simulink model "pivotsimulation"  (R2026a)
settings: Solver=ode15s  StopTime=30  AbsTol=1e-3  EnableMultiTasking=on
undefined symbols (not defined in the file): X, Y, Z
libraries: sm_lib x21, nesl_utility x4
settings Model: Creator=emmak  LastModifiedBy=emmak
settings DebuggingCC: SubsystemReferenceDiagnosticForUnitTest=warning
settings SimscapeCC: SimscapeNominalValues="[{\"value\":\"1\",\"unit\":\"A\"},{\"value\":\"1\",\"unit\":\"bar\"},{\"value\":\"1\",\"unit\":\"cm^2\"},{\"value\":\"1\",\"unit\":\"cm^3/s\"},{\"value\":\"1\",\"unit\":\"kJ/kg\"},{\"value\":\"1\",\"unit\":\"kW\"},{\"value\":\"1\",\"unit\":\"l\"},{\"value\":\"1\",\"unit\":\"N\"},{\"value\":\"1\",\"unit\":\"N*m\"},{\"value\":\"1\",\"unit\":\"V\"}]"

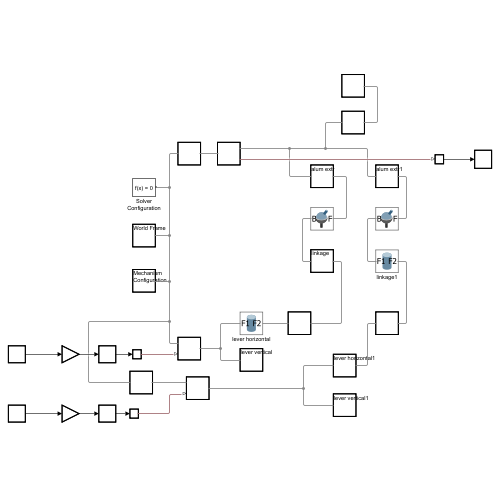
[thumbnail: Simulink's stored preview of the top-level diagram]
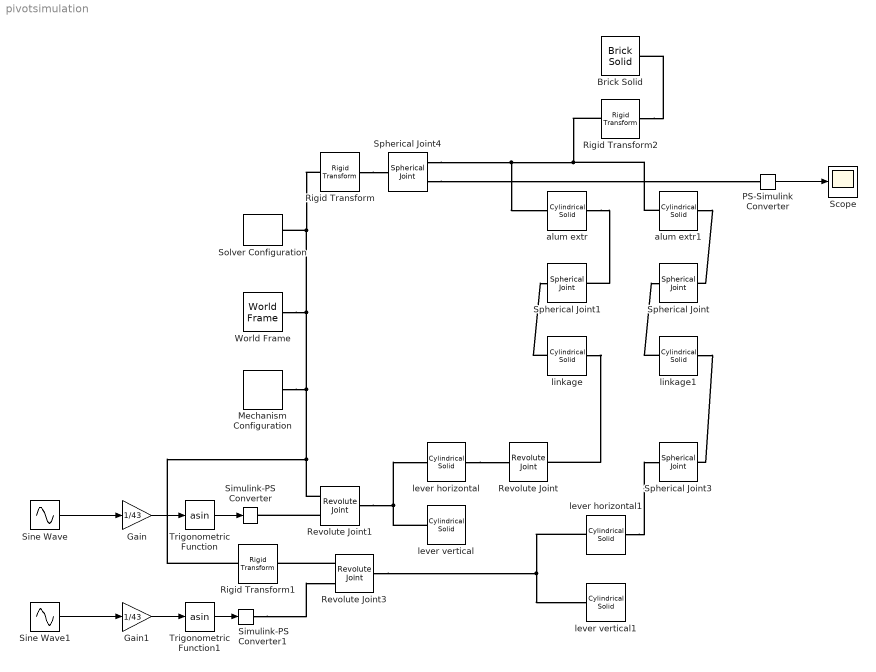
== system pivotsimulation ==
  Brick Solid : sm_lib/Body Elements/Brick Solid  BrickDimensions=[600 10 400]  BrickDimensionsUnits=mm  ExportEntireGeometry=off  InertiaType=CalculateFromGeometry  BasedOnType=Density  Density=1000  DensityUnits=kg/m^3  Mass=1  MassUnits=kg  CenterOfMass=[0 0 0]  CenterOfMassUnits=m  MomentsOfInertia=[1 1 1]  MomentsOfInertiaUnits=kg*m^2  ProductsOfInertia=[0 0 0]  ProductsOfInertiaUnits=kg*m^2  GraphicType=FromGeometry  MarkerShape=Sphere  MarkerSize=10  GraphicVisPropType=SimpleVisualProperties  GraphicDiffuseColor=[0.6471 0.5255 0.3843]  GraphicOpacity=1  GraphicSpecularColor=[0.5 0.5 0.5 1.0]  GraphicAmbientColor=[0.15 0.15 0.15 1.0]  GraphicEmissiveColor=[0.0 0.0 0.0 1.0]  GraphicShininess=75  DoExposeReferenceFrame=on  SerializedFrames=<Frames/>
  Gain : Gain  Gain=1/43
  Gain1 : Gain  Gain=1/43
  Mechanism Configuration : sm_lib/Utilities/Mechanism Configuration  UniformGravity=Constant  GravityVector=[0 -9.80665 0]  GravityVectorUnits=m/s^2  LinearizationDelta=0.001  JointModeTransitionNonlinearIterations=2
  PS-Simulink Converter : nesl_utility/PS-Simulink Converter  PhysicalDomain=network_engine_domain  SubClassName=ps_output  LeftPortType=input  RightPortType=output  PseudoPeriodic=off  Frequencies=[]  VectorFormat=inherit  Unit=inherit  AffineConversion=off
  Revolute Joint : sm_lib/Joints/Revolute Joint  JointMode=Normal  CompositeWrenchDir=FollowerOnBase  CompositeWrenchFrame=BaseFrame  SenseConstraintForce=off  SenseConstraintTorque=off  SenseTotalForce=off  SenseTotalTorque=off  PositionTargetSpecify=off  PositionTargetPriority=High  PositionTargetValue=0  PositionTargetValueUnits=deg  VelocityTargetSpecify=off  VelocityTargetPriority=High  VelocityTargetValue=0  VelocityTargetValueUnits=deg/s  EquilibriumPosition=0  EquilibriumPositionUnits=deg  SpringStiffness=0  SpringStiffnessUnits=N*m/deg  DampingCoefficient=0  DampingCoefficientUnits=N*m/(deg/s)  LowerLimitSpecify=off  LowerLimitBound=-90  LowerLimitBoundUnits=deg  LowerLimitStiffness=1e4  LowerLimitStiffnessUnits=N*m/deg  LowerLimitDamping=10  LowerLimitDampingUnits=N*m/(deg/s)  LowerLimitTransitionRegionWidth=0.1  LowerLimitTransitionRegionWidthUnits=deg  UpperLimitSpecify=off  UpperLimitBound=90  UpperLimitBoundUnits=deg  UpperLimitStiffness=1e4  UpperLimitStiffnessUnits=N*m/deg  UpperLimitDamping=10  UpperLimitDampingUnits=N*m/(deg/s)  UpperLimitTransitionRegionWidth=0.1  UpperLimitTransitionRegionWidthUnits=deg  TorqueActuationMode=NoTorque  MotionActuationMode=ComputedMotion  SensePosition=off  SenseVelocity=off  SenseAcceleration=off  SenseTorqueForce=off  SenseLowerLimitTorqueForce=off  SenseUpperLimitTorqueForce=off
  Revolute Joint1 : sm_lib/Joints/Revolute Joint  JointMode=Normal  CompositeWrenchDir=FollowerOnBase  CompositeWrenchFrame=BaseFrame  SenseConstraintForce=off  SenseConstraintTorque=off  SenseTotalForce=off  SenseTotalTorque=off  PositionTargetSpecify=off  PositionTargetPriority=High  PositionTargetValue=0  PositionTargetValueUnits=deg  VelocityTargetSpecify=off  VelocityTargetPriority=High  VelocityTargetValue=0  VelocityTargetValueUnits=deg/s  EquilibriumPosition=0  EquilibriumPositionUnits=deg  SpringStiffness=0  SpringStiffnessUnits=N*m/deg  DampingCoefficient=0  DampingCoefficientUnits=N*m/(deg/s)  LowerLimitSpecify=off  LowerLimitBound=-90  LowerLimitBoundUnits=deg  LowerLimitStiffness=1e4  LowerLimitStiffnessUnits=N*m/deg  LowerLimitDamping=10  LowerLimitDampingUnits=N*m/(deg/s)  LowerLimitTransitionRegionWidth=0.1  LowerLimitTransitionRegionWidthUnits=deg  UpperLimitSpecify=off  UpperLimitBound=90  UpperLimitBoundUnits=deg  UpperLimitStiffness=1e4  UpperLimitStiffnessUnits=N*m/deg  UpperLimitDamping=10  UpperLimitDampingUnits=N*m/(deg/s)  UpperLimitTransitionRegionWidth=0.1  UpperLimitTransitionRegionWidthUnits=deg  TorqueActuationMode=ComputedTorque  MotionActuationMode=InputMotion  SensePosition=off  SenseVelocity=off  SenseAcceleration=off  SenseTorqueForce=off  SenseLowerLimitTorqueForce=off  SenseUpperLimitTorqueForce=off
  Revolute Joint3 : sm_lib/Joints/Revolute Joint  JointMode=Normal  CompositeWrenchDir=FollowerOnBase  CompositeWrenchFrame=BaseFrame  SenseConstraintForce=off  SenseConstraintTorque=off  SenseTotalForce=off  SenseTotalTorque=off  PositionTargetSpecify=off  PositionTargetPriority=High  PositionTargetValue=0  PositionTargetValueUnits=deg  VelocityTargetSpecify=off  VelocityTargetPriority=High  VelocityTargetValue=0  VelocityTargetValueUnits=deg/s  EquilibriumPosition=0  EquilibriumPositionUnits=deg  SpringStiffness=0  SpringStiffnessUnits=N*m/deg  DampingCoefficient=0  DampingCoefficientUnits=N*m/(deg/s)  LowerLimitSpecify=off  LowerLimitBound=-90  LowerLimitBoundUnits=deg  LowerLimitStiffness=1e4  LowerLimitStiffnessUnits=N*m/deg  LowerLimitDamping=10  LowerLimitDampingUnits=N*m/(deg/s)  LowerLimitTransitionRegionWidth=0.1  LowerLimitTransitionRegionWidthUnits=deg  UpperLimitSpecify=off  UpperLimitBound=90  UpperLimitBoundUnits=deg  UpperLimitStiffness=1e4  UpperLimitStiffnessUnits=N*m/deg  UpperLimitDamping=10  UpperLimitDampingUnits=N*m/(deg/s)  UpperLimitTransitionRegionWidth=0.1  UpperLimitTransitionRegionWidthUnits=deg  TorqueActuationMode=ComputedTorque  MotionActuationMode=InputMotion  SensePosition=off  SenseVelocity=off  SenseAcceleration=off  SenseTorqueForce=off  SenseLowerLimitTorqueForce=off  SenseUpperLimitTorqueForce=off
  Rigid Transform : sm_lib/Frames and Transforms/Rigid Transform  RotationMethod=None  FollAlignAxisA=+X  BaseAlignAxisA=+Y  FollAlignAxisB=+Y  BaseAlignAxisB=+Z  RotationStandardAxis=+Z  RotationAngle=0  RotationAngleUnits=deg  RotationArbitraryAxis=[0 0 1]  RotationSequenceAxes=FollowerAxes  RotationSequence=XYX  RotationSequenceAngles=[0 0 0]  RotationSequenceAnglesUnits=deg  RotationMatrix=[1 0 0;0 1 0;0 0 1]  Quaternion=[1 0 0 0]  TranslationMethod=Cartesian  TranslationCartesianOffset=[265 91 0]  TranslationCartesianOffsetUnits=mm  TranslationStandardAxis=+Z  TranslationStandardOffset=0  TranslationStandardOffsetUnits=m  TranslationROffset=0  TranslationROffsetUnits=m  TranslationThetaOffset=0  TranslationThetaOffsetUnits=deg  TranslationZOffset=0  TranslationZOffsetUnits=m
  Rigid Transform1 : sm_lib/Frames and Transforms/Rigid Transform  RotationMethod=None  FollAlignAxisA=+X  BaseAlignAxisA=+Y  FollAlignAxisB=+Y  BaseAlignAxisB=+Z  RotationStandardAxis=+Z  RotationAngle=0  RotationAngleUnits=deg  RotationArbitraryAxis=[0 0 1]  RotationSequenceAxes=FollowerAxes  RotationSequence=XYX  RotationSequenceAngles=[0 0 0]  RotationSequenceAnglesUnits=deg  RotationMatrix=[1 0 0;0 1 0;0 0 1]  Quaternion=[1 0 0 0]  TranslationMethod=Cartesian  TranslationCartesianOffset=[285 0 146]  TranslationCartesianOffsetUnits=mm  TranslationStandardAxis=+Z  TranslationStandardOffset=0  TranslationStandardOffsetUnits=m  TranslationROffset=0  TranslationROffsetUnits=m  TranslationThetaOffset=0  TranslationThetaOffsetUnits=deg  TranslationZOffset=0  TranslationZOffsetUnits=m
  Rigid Transform2 : sm_lib/Frames and Transforms/Rigid Transform  RotationMethod=None  FollAlignAxisA=+X  BaseAlignAxisA=+Y  FollAlignAxisB=+Y  BaseAlignAxisB=+Z  RotationStandardAxis=+Z  RotationAngle=0  RotationAngleUnits=deg  RotationArbitraryAxis=[0 0 1]  RotationSequenceAxes=FollowerAxes  RotationSequence=XYX  RotationSequenceAngles=[0 0 0]  RotationSequenceAnglesUnits=deg  RotationMatrix=[1 0 0;0 1 0;0 0 1]  Quaternion=[1 0 0 0]  TranslationMethod=Cartesian  TranslationCartesianOffset=[0 10 0]  TranslationCartesianOffsetUnits=mm  TranslationStandardAxis=+Z  TranslationStandardOffset=0  TranslationStandardOffsetUnits=m  TranslationROffset=0  TranslationROffsetUnits=m  TranslationThetaOffset=0  TranslationThetaOffsetUnits=deg  TranslationZOffset=0  TranslationZOffsetUnits=m
  Scope : Scope
      settings: ActiveDisplayYMinimum=-0.3302984984477686  ActiveDisplayYMaximum=0.32500944706024004
  Simulink-PS Converter : nesl_utility/Simulink-PS Converter  PhysicalDomain=network_engine_domain  SubClassName=ps_input  LeftPortType=input  RightPortType=output  PseudoPeriodic=off  Frequencies=[]  NoiseDistribution=none  NoiseParameters=[]  Unit=1  AffineConversion=off  FilteringAndDerivatives=filter  SimscapeFilterOrder=2  InputFilterTimeConstant=0.001  UdotUserProvided=0
  Simulink-PS Converter1 : nesl_utility/Simulink-PS Converter  PhysicalDomain=network_engine_domain  SubClassName=ps_input  LeftPortType=input  RightPortType=output  PseudoPeriodic=off  Frequencies=[]  NoiseDistribution=none  NoiseParameters=[]  Unit=1  AffineConversion=off  FilteringAndDerivatives=filter  SimscapeFilterOrder=2  InputFilterTimeConstant=0.001  UdotUserProvided=0
  Sine Wave : Sin  Amplitude=25  SampleTime=0
  Sine Wave1 : Sin  Amplitude=25  Frequency=1.5  Phase=(pi)  SampleTime=0
  Solver Configuration : nesl_utility/Solver Configuration  PhysicalDomain=network_engine_domain  SubClassName=solver  LeftPortType=input  RightPortType=generic  Tones=[]  Harmonics=[]  SimulateNoise=off  Profile=off  UseLocalSampling=off  EnableSwitchedLinearOptims=on  FrequencyDomain=off  UseCCode=off  RelTol=0.001  AbsTol=1e-06  MinStep=1e-09  ToWorkspace=off  RevertToSquareIcSolve=off  NumHomotopyIterations=100  PhasorMode=off  PhasorModeNumHarmonics=1  ConsistencySolver=NEWTON_XTOL_AFTER_FTOL  CanonicalOrdering=UNORDERED  OptimizeIntermediates=UNOPTIMIZED  IndexReductionMethod=DerivativeReplacement  DoDC=off  ResidualTolerance=1e-09  ConsistencyTolSource=GLOBAL  ConsistencyAbsTol=0.001  ConsistencyRelTol=0.001  ConsistencyTolFactor=0.001  UseLocalSolver=off  LocalSolverChoice=NE_BACKWARD_EULER_ADVANCER  ResolveIndetEquations=on  FunctionEvalNumThread=1  LocalSolverSampleTime=0.001  DoFixedCost=off  MaxNonlinIter=3  MaxModeIter=2  ComputeImpulses=off  ImpulseIterations=2  LinearAlgebra=Sparse  LinearAlgebraNumThread=0  EquationFormulation=NE_TIME_EF  DelaysMemoryBudget=1024  AutomaticFiltering=on  FilteringTimeConstant=0.001  PartitionStorageMethod=AS_NEEDED  PartitionMemoryBudget=1024  PartitionMethod=FAST  MultibodyUseLocalSolver=off  MultibodyLocalSolverChoice=ODE1  MultibodyLocalSolverSampleTime=0.001
  Spherical Joint : sm_lib/Joints/Spherical Joint  JointMode=Normal  CompositeWrenchDir=FollowerOnBase  CompositeWrenchFrame=BaseFrame  SenseConstraintForce=off  SenseConstraintTorque=off  SenseTotalForce=off  SenseTotalTorque=off  PositionTargetSpecify=off  PositionTargetPriority=High  PositionTargetRotationMethod=None  PositionTargetFollAlignAxisA=+X  PositionTargetBaseAlignAxisA=+Y  PositionTargetFollAlignAxisB=+Y  PositionTargetBaseAlignAxisB=+Z  PositionTargetRotationStandardAxis=+Z  PositionTargetRotationAngle=0  PositionTargetRotationAngleUnits=deg  PositionTargetRotationArbitraryAxis=[0 0 1]  PositionTargetRotationSequenceAxes=FollowerAxes  PositionTargetRotationSequence=XYX  PositionTargetRotationSequenceAngles=[0 0 0]  PositionTargetRotationSequenceAnglesUnits=deg  PositionTargetRotationMatrix=[1 0 0;0 1 0;0 0 1]  PositionTargetQuaternion=[1 0 0 0]  VelocityTargetSpecify=off  VelocityTargetPriority=High  VelocityTargetValue=[0 0 0]  VelocityTargetValueUnits=deg/s  VelocityTargetInFollowerFrame=on  EqPosRotationMethod=None  EqPosFollAlignAxisA=+X  EqPosBaseAlignAxisA=+Y  EqPosFollAlignAxisB=+Y  EqPosBaseAlignAxisB=+Z  EqPosRotationStandardAxis=+Z  EqPosRotationAngle=0  EqPosRotationAngleUnits=deg  EqPosRotationArbitraryAxis=[0 0 1]  EqPosRotationSequenceAxes=FollowerAxes  EqPosRotationSequence=XYX  EqPosRotationSequenceAngles=[0 0 0]  EqPosRotationSequenceAnglesUnits=deg  EqPosRotationMatrix=[1 0 0;0 1 0;0 0 1]  EqPosQuaternion=[1 0 0 0]  SpringStiffness=0  SpringStiffnessUnits=N*m/deg  DampingCoefficient=0  DampingCoefficientUnits=N*m/(deg/s)  LowerLimitSpecify=off  LowerLimitBound=15  LowerLimitBoundUnits=deg  LowerLimitStiffness=1e4  LowerLimitStiffnessUnits=N*m/deg  LowerLimitDamping=10  LowerLimitDampingUnits=N*m/(deg/s)  LowerLimitTransitionRegionWidth=0.1  LowerLimitTransitionRegionWidthUnits=deg  UpperLimitSpecify=off  UpperLimitBound=45  UpperLimitBoundUnits=deg  UpperLimitStiffness=1e4  UpperLimitStiffnessUnits=N*m/deg  UpperLimitDamping=10  UpperLimitDampingUnits=N*m/(deg/s)  UpperLimitTransitionRegionWidth=0.1  UpperLimitTransitionRegionWidthUnits=deg  TorqueActuationMode=NoTorque  ActuateTorqueX=off  ActuateTorqueY=off  ActuateTorqueZ=off  ActuateTorque=off  ActuationFrame=BaseFrame  SensePosition=off  SenseVelocityX=off  SenseVelocityY=off  SenseVelocityZ=off  SenseVelocity=off  SenseAccelerationX=off  SenseAccelerationY=off  SenseAccelerationZ=off  SenseAcceleration=off  SenseLowerLimitTorqueMag=off  SenseUpperLimitTorqueMag=off  SensingFrame=BaseFrame
  Spherical Joint1 : sm_lib/Joints/Spherical Joint  JointMode=Normal  CompositeWrenchDir=FollowerOnBase  CompositeWrenchFrame=BaseFrame  SenseConstraintForce=off  SenseConstraintTorque=off  SenseTotalForce=off  SenseTotalTorque=off  PositionTargetSpecify=off  PositionTargetPriority=High  PositionTargetRotationMethod=None  PositionTargetFollAlignAxisA=+X  PositionTargetBaseAlignAxisA=+Y  PositionTargetFollAlignAxisB=+Y  PositionTargetBaseAlignAxisB=+Z  PositionTargetRotationStandardAxis=+Z  PositionTargetRotationAngle=0  PositionTargetRotationAngleUnits=deg  PositionTargetRotationArbitraryAxis=[0 0 1]  PositionTargetRotationSequenceAxes=FollowerAxes  PositionTargetRotationSequence=XYX  PositionTargetRotationSequenceAngles=[0 0 0]  PositionTargetRotationSequenceAnglesUnits=deg  PositionTargetRotationMatrix=[1 0 0;0 1 0;0 0 1]  PositionTargetQuaternion=[1 0 0 0]  VelocityTargetSpecify=off  VelocityTargetPriority=High  VelocityTargetValue=[0 0 0]  VelocityTargetValueUnits=deg/s  VelocityTargetInFollowerFrame=on  EqPosRotationMethod=None  EqPosFollAlignAxisA=+X  EqPosBaseAlignAxisA=+Y  EqPosFollAlignAxisB=+Y  EqPosBaseAlignAxisB=+Z  EqPosRotationStandardAxis=+Z  EqPosRotationAngle=0  EqPosRotationAngleUnits=deg  EqPosRotationArbitraryAxis=[0 0 1]  EqPosRotationSequenceAxes=FollowerAxes  EqPosRotationSequence=XYX  EqPosRotationSequenceAngles=[0 0 0]  EqPosRotationSequenceAnglesUnits=deg  EqPosRotationMatrix=[1 0 0;0 1 0;0 0 1]  EqPosQuaternion=[1 0 0 0]  SpringStiffness=0  SpringStiffnessUnits=N*m/deg  DampingCoefficient=0  DampingCoefficientUnits=N*m/(deg/s)  LowerLimitSpecify=off  LowerLimitBound=15  LowerLimitBoundUnits=deg  LowerLimitStiffness=1e4  LowerLimitStiffnessUnits=N*m/deg  LowerLimitDamping=10  LowerLimitDampingUnits=N*m/(deg/s)  LowerLimitTransitionRegionWidth=0.1  LowerLimitTransitionRegionWidthUnits=deg  UpperLimitSpecify=off  UpperLimitBound=45  UpperLimitBoundUnits=deg  UpperLimitStiffness=1e4  UpperLimitStiffnessUnits=N*m/deg  UpperLimitDamping=10  UpperLimitDampingUnits=N*m/(deg/s)  UpperLimitTransitionRegionWidth=0.1  UpperLimitTransitionRegionWidthUnits=deg  TorqueActuationMode=NoTorque  ActuateTorqueX=off  ActuateTorqueY=off  ActuateTorqueZ=off  ActuateTorque=off  ActuationFrame=BaseFrame  SensePosition=off  SenseVelocityX=off  SenseVelocityY=off  SenseVelocityZ=off  SenseVelocity=off  SenseAccelerationX=off  SenseAccelerationY=off  SenseAccelerationZ=off  SenseAcceleration=off  SenseLowerLimitTorqueMag=off  SenseUpperLimitTorqueMag=off  SensingFrame=BaseFrame
  Spherical Joint3 : sm_lib/Joints/Spherical Joint  JointMode=Normal  CompositeWrenchDir=FollowerOnBase  CompositeWrenchFrame=BaseFrame  SenseConstraintForce=off  SenseConstraintTorque=off  SenseTotalForce=off  SenseTotalTorque=off  PositionTargetSpecify=off  PositionTargetPriority=High  PositionTargetRotationMethod=None  PositionTargetFollAlignAxisA=+X  PositionTargetBaseAlignAxisA=+Y  PositionTargetFollAlignAxisB=+Y  PositionTargetBaseAlignAxisB=+Z  PositionTargetRotationStandardAxis=+Z  PositionTargetRotationAngle=0  PositionTargetRotationAngleUnits=deg  PositionTargetRotationArbitraryAxis=[0 0 1]  PositionTargetRotationSequenceAxes=FollowerAxes  PositionTargetRotationSequence=XYX  PositionTargetRotationSequenceAngles=[0 0 0]  PositionTargetRotationSequenceAnglesUnits=deg  PositionTargetRotationMatrix=[1 0 0;0 1 0;0 0 1]  PositionTargetQuaternion=[1 0 0 0]  VelocityTargetSpecify=off  VelocityTargetPriority=High  VelocityTargetValue=[0 0 0]  VelocityTargetValueUnits=deg/s  VelocityTargetInFollowerFrame=on  EqPosRotationMethod=None  EqPosFollAlignAxisA=+X  EqPosBaseAlignAxisA=+Y  EqPosFollAlignAxisB=+Y  EqPosBaseAlignAxisB=+Z  EqPosRotationStandardAxis=+Z  EqPosRotationAngle=0  EqPosRotationAngleUnits=deg  EqPosRotationArbitraryAxis=[0 0 1]  EqPosRotationSequenceAxes=FollowerAxes  EqPosRotationSequence=XYX  EqPosRotationSequenceAngles=[0 0 0]  EqPosRotationSequenceAnglesUnits=deg  EqPosRotationMatrix=[1 0 0;0 1 0;0 0 1]  EqPosQuaternion=[1 0 0 0]  SpringStiffness=0  SpringStiffnessUnits=N*m/deg  DampingCoefficient=0  DampingCoefficientUnits=N*m/(deg/s)  LowerLimitSpecify=off  LowerLimitBound=15  LowerLimitBoundUnits=deg  LowerLimitStiffness=1e4  LowerLimitStiffnessUnits=N*m/deg  LowerLimitDamping=10  LowerLimitDampingUnits=N*m/(deg/s)  LowerLimitTransitionRegionWidth=0.1  LowerLimitTransitionRegionWidthUnits=deg  UpperLimitSpecify=off  UpperLimitBound=45  UpperLimitBoundUnits=deg  UpperLimitStiffness=1e4  UpperLimitStiffnessUnits=N*m/deg  UpperLimitDamping=10  UpperLimitDampingUnits=N*m/(deg/s)  UpperLimitTransitionRegionWidth=0.1  UpperLimitTransitionRegionWidthUnits=deg  TorqueActuationMode=NoTorque  ActuateTorqueX=off  ActuateTorqueY=off  ActuateTorqueZ=off  ActuateTorque=off  ActuationFrame=BaseFrame  SensePosition=off  SenseVelocityX=off  SenseVelocityY=off  SenseVelocityZ=off  SenseVelocity=off  SenseAccelerationX=off  SenseAccelerationY=off  SenseAccelerationZ=off  SenseAcceleration=off  SenseLowerLimitTorqueMag=off  SenseUpperLimitTorqueMag=off  SensingFrame=BaseFrame
  Spherical Joint4 : sm_lib/Joints/Spherical Joint  JointMode=Normal  CompositeWrenchDir=FollowerOnBase  CompositeWrenchFrame=BaseFrame  SenseConstraintForce=off  SenseConstraintTorque=off  SenseTotalForce=off  SenseTotalTorque=off  PositionTargetSpecify=off  PositionTargetPriority=High  PositionTargetRotationMethod=None  PositionTargetFollAlignAxisA=+X  PositionTargetBaseAlignAxisA=+Y  PositionTargetFollAlignAxisB=+Y  PositionTargetBaseAlignAxisB=+Z  PositionTargetRotationStandardAxis=+Z  PositionTargetRotationAngle=0  PositionTargetRotationAngleUnits=deg  PositionTargetRotationArbitraryAxis=[0 0 1]  PositionTargetRotationSequenceAxes=FollowerAxes  PositionTargetRotationSequence=XYX  PositionTargetRotationSequenceAngles=[0 0 0]  PositionTargetRotationSequenceAnglesUnits=deg  PositionTargetRotationMatrix=[1 0 0;0 1 0;0 0 1]  PositionTargetQuaternion=[1 0 0 0]  VelocityTargetSpecify=off  VelocityTargetPriority=High  VelocityTargetValue=[0 0 0]  VelocityTargetValueUnits=deg/s  VelocityTargetInFollowerFrame=on  EqPosRotationMethod=None  EqPosFollAlignAxisA=+X  EqPosBaseAlignAxisA=+Y  EqPosFollAlignAxisB=+Y  EqPosBaseAlignAxisB=+Z  EqPosRotationStandardAxis=+Z  EqPosRotationAngle=0  EqPosRotationAngleUnits=deg  EqPosRotationArbitraryAxis=[0 0 1]  EqPosRotationSequenceAxes=FollowerAxes  EqPosRotationSequence=XYX  EqPosRotationSequenceAngles=[0 0 0]  EqPosRotationSequenceAnglesUnits=deg  EqPosRotationMatrix=[1 0 0;0 1 0;0 0 1]  EqPosQuaternion=[1 0 0 0]  SpringStiffness=0  SpringStiffnessUnits=N*m/deg  DampingCoefficient=0  DampingCoefficientUnits=N*m/(deg/s)  LowerLimitSpecify=off  LowerLimitBound=15  LowerLimitBoundUnits=deg  LowerLimitStiffness=1e4  LowerLimitStiffnessUnits=N*m/deg  LowerLimitDamping=10  LowerLimitDampingUnits=N*m/(deg/s)  LowerLimitTransitionRegionWidth=0.1  LowerLimitTransitionRegionWidthUnits=deg  UpperLimitSpecify=off  UpperLimitBound=45  UpperLimitBoundUnits=deg  UpperLimitStiffness=1e4  UpperLimitStiffnessUnits=N*m/deg  UpperLimitDamping=10  UpperLimitDampingUnits=N*m/(deg/s)  UpperLimitTransitionRegionWidth=0.1  UpperLimitTransitionRegionWidthUnits=deg  TorqueActuationMode=NoTorque  ActuateTorqueX=off  ActuateTorqueY=off  ActuateTorqueZ=off  ActuateTorque=off  ActuationFrame=BaseFrame  SensePosition=on  SenseVelocityX=off  SenseVelocityY=off  SenseVelocityZ=off  SenseVelocity=off  SenseAccelerationX=off  SenseAccelerationY=off  SenseAccelerationZ=off  SenseAcceleration=off  SenseLowerLimitTorqueMag=off  SenseUpperLimitTorqueMag=off  SensingFrame=BaseFrame
  Trigonometric Function : Trigonometry  Operator=asin
  Trigonometric Function1 : Trigonometry  Operator=asin
  World Frame : sm_lib/Frames and Transforms/World Frame
  alum extr : sm_lib/Body Elements/Cylindrical Solid  CylinderRadius=5  CylinderRadiusUnits=mm  CylinderLength=245  CylinderLengthUnits=mm  ExportEntireGeometry=off  InertiaType=CalculateFromGeometry  BasedOnType=Density  Density=1000  DensityUnits=kg/m^3  Mass=1  MassUnits=kg  CenterOfMass=[0 0 0]  CenterOfMassUnits=m  MomentsOfInertia=[1 1 1]  MomentsOfInertiaUnits=kg*m^2  ProductsOfInertia=[0 0 0]  ProductsOfInertiaUnits=kg*m^2  GraphicType=FromGeometry  MarkerShape=Sphere  MarkerSize=10  GraphicVisPropType=SimpleVisualProperties  GraphicDiffuseColor=[0.5 0.5 0.5]  GraphicOpacity=1  GraphicSpecularColor=[0.5 0.5 0.5 1.0]  GraphicAmbientColor=[0.15 0.15 0.15 1.0]  GraphicEmissiveColor=[0.0 0.0 0.0 1.0]  GraphicShininess=75  DoExposeReferenceFrame=off  SerializedFrames=<Frames><Frame><Id>Frame1</Id><Value><Name>F1</Name><Origin><Source>GeometricFeature</Source><FeatureName>bottom surface</FeatureName></Origin><PrimaryAxis><DefinedDirection>-X</DefinedDirection><Source>ReferenceFrame</Source><SourceDirection>+Z</SourceDirection><FeatureName></FeatureName></PrimaryAxis><SecondaryAxis><DefinedDirection>+Y</DefinedDirection><Source>ReferenceFrame</Source><SourceDirection>+Y</SourceDirection><FeatureName></FeatureName></SecondaryAxis></Value></Frame><Frame><Id>Frame2</Id><Value><Name>F2</Name><Origin><Source>GeometricFeature</Source><FeatureName>top curve</FeatureName></Origin><PrimaryAxis><DefinedDirection>+Y</DefinedDirection><Source>ReferenceFrame</Source><SourceDirection>+Y</SourceDirection><FeatureName></FeatureName></PrimaryAxis><SecondaryAxis><DefinedDirection>+X</DefinedDirection><Source>ReferenceFrame</Source><SourceDirection>-Z</SourceDirection><FeatureName></FeatureName></SecondaryAxis></Value></Frame></Frames>
  alum extr1 : sm_lib/Body Elements/Cylindrical Solid  CylinderRadius=5  CylinderRadiusUnits=mm  CylinderLength=146  CylinderLengthUnits=mm  ExportEntireGeometry=off  InertiaType=CalculateFromGeometry  BasedOnType=Density  Density=1000  DensityUnits=kg/m^3  Mass=1  MassUnits=kg  CenterOfMass=[0 0 0]  CenterOfMassUnits=m  MomentsOfInertia=[1 1 1]  MomentsOfInertiaUnits=kg*m^2  ProductsOfInertia=[0 0 0]  ProductsOfInertiaUnits=kg*m^2  GraphicType=FromGeometry  MarkerShape=Sphere  MarkerSize=10  GraphicVisPropType=SimpleVisualProperties  GraphicDiffuseColor=[0.5 0.5 0.5]  GraphicOpacity=1  GraphicSpecularColor=[0.5 0.5 0.5 1.0]  GraphicAmbientColor=[0.15 0.15 0.15 1.0]  GraphicEmissiveColor=[0.0 0.0 0.0 1.0]  GraphicShininess=75  DoExposeReferenceFrame=off  SerializedFrames=<Frames><Frame><Id>Frame1</Id><Value><Name>F1</Name><Origin><Source>GeometricFeature</Source><FeatureName>bottom surface</FeatureName></Origin><PrimaryAxis><DefinedDirection>+X</DefinedDirection><Source>ReferenceFrame</Source><SourceDirection>+X</SourceDirection><FeatureName></FeatureName></PrimaryAxis><SecondaryAxis><DefinedDirection>+Y</DefinedDirection><Source>ReferenceFrame</Source><SourceDirection>+Y</SourceDirection><FeatureName></FeatureName></SecondaryAxis></Value></Frame><Frame><Id>Frame2</Id><Value><Name>F2</Name><Origin><Source>GeometricFeature</Source><FeatureName>top curve</FeatureName></Origin><PrimaryAxis><DefinedDirection>+Y</DefinedDirection><Source>ReferenceFrame</Source><SourceDirection>+Y</SourceDirection><FeatureName></FeatureName></PrimaryAxis><SecondaryAxis><DefinedDirection>+X</DefinedDirection><Source>ReferenceFrame</Source><SourceDirection>+X</SourceDirection><FeatureName></FeatureName></SecondaryAxis></Value></Frame></Frames>
  lever horizontal : sm_lib/Body Elements/Cylindrical Solid  CylinderRadius=5  CylinderRadiusUnits=mm  CylinderLength=43  CylinderLengthUnits=mm  ExportEntireGeometry=off  InertiaType=CalculateFromGeometry  BasedOnType=Density  Density=1000  DensityUnits=kg/m^3  Mass=1  MassUnits=kg  CenterOfMass=[0 0 0]  CenterOfMassUnits=m  MomentsOfInertia=[1 1 1]  MomentsOfInertiaUnits=kg*m^2  ProductsOfInertia=[0 0 0]  ProductsOfInertiaUnits=kg*m^2  GraphicType=FromGeometry  MarkerShape=Sphere  MarkerSize=10  GraphicVisPropType=SimpleVisualProperties  GraphicDiffuseColor=[0.5 0.5 0.5]  GraphicOpacity=1  GraphicSpecularColor=[0.5 0.5 0.5 1.0]  GraphicAmbientColor=[0.15 0.15 0.15 1.0]  GraphicEmissiveColor=[0.0 0.0 0.0 1.0]  GraphicShininess=75  DoExposeReferenceFrame=off  SerializedFrames=<Frames><Frame><Id>Frame1</Id><Value><Name>F1</Name><Origin><Source>GeometricFeature</Source><FeatureName>top surface</FeatureName></Origin><PrimaryAxis><DefinedDirection>+Z</DefinedDirection><Source>ReferenceFrame</Source><SourceDirection>+X</SourceDirection><FeatureName></FeatureName></PrimaryAxis><SecondaryAxis><DefinedDirection>+Y</DefinedDirection><Source>ReferenceFrame</Source><SourceDirection>+Y</SourceDirection><FeatureName></FeatureName></SecondaryAxis></Value></Frame><Frame><Id>Frame2</Id><Value><Name>F2</Name><Origin><Source>GeometricFeature</Source><FeatureName>bottom surface</FeatureName></Origin><PrimaryAxis><DefinedDirection>+Y</DefinedDirection><Source>ReferenceFrame</Source><SourceDirection>+Y</SourceDirection><FeatureName></FeatureName></PrimaryAxis><SecondaryAxis><DefinedDirection>+Z</DefinedDirection><Source>ReferenceFrame</Source><SourceDirection>+X</SourceDirection><FeatureName></FeatureName></SecondaryAxis></Value></Frame></Frames>
  lever horizontal1 : sm_lib/Body Elements/Cylindrical Solid  CylinderRadius=5  CylinderRadiusUnits=mm  CylinderLength=43  CylinderLengthUnits=mm  ExportEntireGeometry=off  InertiaType=CalculateFromGeometry  BasedOnType=Density  Density=1000  DensityUnits=kg/m^3  Mass=1  MassUnits=kg  CenterOfMass=[0 0 0]  CenterOfMassUnits=m  MomentsOfInertia=[1 1 1]  MomentsOfInertiaUnits=kg*m^2  ProductsOfInertia=[0 0 0]  ProductsOfInertiaUnits=kg*m^2  GraphicType=FromGeometry  MarkerShape=Sphere  MarkerSize=10  GraphicVisPropType=SimpleVisualProperties  GraphicDiffuseColor=[0.5 0.5 0.5]  GraphicOpacity=1  GraphicSpecularColor=[0.5 0.5 0.5 1.0]  GraphicAmbientColor=[0.15 0.15 0.15 1.0]  GraphicEmissiveColor=[0.0 0.0 0.0 1.0]  GraphicShininess=75  DoExposeReferenceFrame=off  SerializedFrames=<Frames><Frame><Id>Frame1</Id><Value><Name>F1</Name><Origin><Source>GeometricFeature</Source><FeatureName>top surface</FeatureName></Origin><PrimaryAxis><DefinedDirection>+Z</DefinedDirection><Source>ReferenceFrame</Source><SourceDirection>+X</SourceDirection><FeatureName></FeatureName></PrimaryAxis><SecondaryAxis><DefinedDirection>+Y</DefinedDirection><Source>ReferenceFrame</Source><SourceDirection>+Y</SourceDirection><FeatureName></FeatureName></SecondaryAxis></Value></Frame><Frame><Id>Frame2</Id><Value><Name>F2</Name><Origin><Source>GeometricFeature</Source><FeatureName>bottom surface</FeatureName></Origin><PrimaryAxis><DefinedDirection>+Y</DefinedDirection><Source>ReferenceFrame</Source><SourceDirection>+Y</SourceDirection><FeatureName></FeatureName></PrimaryAxis><SecondaryAxis><DefinedDirection>+Z</DefinedDirection><Source>ReferenceFrame</Source><SourceDirection>+X</SourceDirection><FeatureName></FeatureName></SecondaryAxis></Value></Frame></Frames>
  lever vertical : sm_lib/Body Elements/Cylindrical Solid  CylinderRadius=5  CylinderRadiusUnits=mm  CylinderLength=43  CylinderLengthUnits=mm  ExportEntireGeometry=off  InertiaType=CalculateFromGeometry  BasedOnType=Density  Density=1000  DensityUnits=kg/m^3  Mass=1  MassUnits=kg  CenterOfMass=[0 0 0]  CenterOfMassUnits=m  MomentsOfInertia=[1 1 1]  MomentsOfInertiaUnits=kg*m^2  ProductsOfInertia=[0 0 0]  ProductsOfInertiaUnits=kg*m^2  GraphicType=FromGeometry  MarkerShape=Sphere  MarkerSize=10  GraphicVisPropType=SimpleVisualProperties  GraphicDiffuseColor=[0.5 0.5 0.5]  GraphicOpacity=1  GraphicSpecularColor=[0.5 0.5 0.5 1.0]  GraphicAmbientColor=[0.15 0.15 0.15 1.0]  GraphicEmissiveColor=[0.0 0.0 0.0 1.0]  GraphicShininess=75  DoExposeReferenceFrame=off  SerializedFrames=<Frames><Frame><Id>Frame1</Id><Value><Name>F1</Name><Origin><Source>GeometricFeature</Source><FeatureName>top surface</FeatureName></Origin><PrimaryAxis><DefinedDirection>+Y</DefinedDirection><Source>ReferenceFrame</Source><SourceDirection>+Z</SourceDirection><FeatureName>top curve</FeatureName></PrimaryAxis><SecondaryAxis><DefinedDirection>+X</DefinedDirection><Source>ReferenceFrame</Source><SourceDirection>+Y</SourceDirection><FeatureName></FeatureName></SecondaryAxis></Value></Frame></Frames>
  lever vertical1 : sm_lib/Body Elements/Cylindrical Solid  CylinderRadius=5  CylinderRadiusUnits=mm  CylinderLength=43  CylinderLengthUnits=mm  ExportEntireGeometry=off  InertiaType=CalculateFromGeometry  BasedOnType=Density  Density=1000  DensityUnits=kg/m^3  Mass=1  MassUnits=kg  CenterOfMass=[0 0 0]  CenterOfMassUnits=m  MomentsOfInertia=[1 1 1]  MomentsOfInertiaUnits=kg*m^2  ProductsOfInertia=[0 0 0]  ProductsOfInertiaUnits=kg*m^2  GraphicType=FromGeometry  MarkerShape=Sphere  MarkerSize=10  GraphicVisPropType=SimpleVisualProperties  GraphicDiffuseColor=[0.5 0.5 0.5]  GraphicOpacity=1  GraphicSpecularColor=[0.5 0.5 0.5 1.0]  GraphicAmbientColor=[0.15 0.15 0.15 1.0]  GraphicEmissiveColor=[0.0 0.0 0.0 1.0]  GraphicShininess=75  DoExposeReferenceFrame=off  SerializedFrames=<Frames><Frame><Id>Frame1</Id><Value><Name>F1</Name><Origin><Source>GeometricFeature</Source><FeatureName>top surface</FeatureName></Origin><PrimaryAxis><DefinedDirection>+Y</DefinedDirection><Source>ReferenceFrame</Source><SourceDirection>+Z</SourceDirection><FeatureName>top curve</FeatureName></PrimaryAxis><SecondaryAxis><DefinedDirection>+X</DefinedDirection><Source>ReferenceFrame</Source><SourceDirection>+Y</SourceDirection><FeatureName></FeatureName></SecondaryAxis></Value></Frame></Frames>
  linkage : sm_lib/Body Elements/Cylindrical Solid  CylinderRadius=5  CylinderRadiusUnits=mm  CylinderLength=93.86  CylinderLengthUnits=mm  ExportEntireGeometry=off  InertiaType=CalculateFromGeometry  BasedOnType=Density  Density=1000  DensityUnits=kg/m^3  Mass=1  MassUnits=kg  CenterOfMass=[0 0 0]  CenterOfMassUnits=m  MomentsOfInertia=[1 1 1]  MomentsOfInertiaUnits=kg*m^2  ProductsOfInertia=[0 0 0]  ProductsOfInertiaUnits=kg*m^2  GraphicType=FromGeometry  MarkerShape=Sphere  MarkerSize=10  GraphicVisPropType=SimpleVisualProperties  GraphicDiffuseColor=[1 0 0]  GraphicOpacity=1  GraphicSpecularColor=[0.5 0.5 0.5 1.0]  GraphicAmbientColor=[0.15 0.15 0.15 1.0]  GraphicEmissiveColor=[0.0 0.0 0.0 1.0]  GraphicShininess=75  DoExposeReferenceFrame=off  SerializedFrames=<Frames><Frame><Id>Frame1</Id><Value><Name>F1</Name><Origin><Source>GeometricFeature</Source><FeatureName>top surface</FeatureName></Origin><PrimaryAxis><DefinedDirection>+Y</DefinedDirection><Source>ReferenceFrame</Source><SourceDirection>+Z</SourceDirection><FeatureName></FeatureName></PrimaryAxis><SecondaryAxis><DefinedDirection>+X</DefinedDirection><Source>ReferenceFrame</Source><SourceDirection>+Y</SourceDirection><FeatureName></FeatureName></SecondaryAxis></Value></Frame><Frame><Id>Frame2</Id><Value><Name>F2</Name><Origin><Source>GeometricFeature</Source><FeatureName>bottom surface</FeatureName></Origin><PrimaryAxis><DefinedDirection>+Y</DefinedDirection><Source>ReferenceFrame</Source><SourceDirection>+Z</SourceDirection><FeatureName></FeatureName></PrimaryAxis><SecondaryAxis><DefinedDirection>+X</DefinedDirection><Source>ReferenceFrame</Source><SourceDirection>+Y</SourceDirection><FeatureName></FeatureName></SecondaryAxis></Value></Frame></Frames>
  linkage1 : sm_lib/Body Elements/Cylindrical Solid  CylinderRadius=5  CylinderRadiusUnits=mm  CylinderLength=93.86  CylinderLengthUnits=mm  ExportEntireGeometry=off  InertiaType=CalculateFromGeometry  BasedOnType=Density  Density=1000  DensityUnits=kg/m^3  Mass=1  MassUnits=kg  CenterOfMass=[0 0 0]  CenterOfMassUnits=m  MomentsOfInertia=[1 1 1]  MomentsOfInertiaUnits=kg*m^2  ProductsOfInertia=[0 0 0]  ProductsOfInertiaUnits=kg*m^2  GraphicType=FromGeometry  MarkerShape=Sphere  MarkerSize=10  GraphicVisPropType=SimpleVisualProperties  GraphicDiffuseColor=[1 0 0]  GraphicOpacity=1  GraphicSpecularColor=[0.5 0.5 0.5 1.0]  GraphicAmbientColor=[0.15 0.15 0.15 1.0]  GraphicEmissiveColor=[0.0 0.0 0.0 1.0]  GraphicShininess=75  DoExposeReferenceFrame=off  SerializedFrames=<Frames><Frame><Id>Frame1</Id><Value><Name>F1</Name><Origin><Source>GeometricFeature</Source><FeatureName>top surface</FeatureName></Origin><PrimaryAxis><DefinedDirection>+Y</DefinedDirection><Source>ReferenceFrame</Source><SourceDirection>+Z</SourceDirection><FeatureName></FeatureName></PrimaryAxis><SecondaryAxis><DefinedDirection>+X</DefinedDirection><Source>ReferenceFrame</Source><SourceDirection>+Y</SourceDirection><FeatureName></FeatureName></SecondaryAxis></Value></Frame><Frame><Id>Frame2</Id><Value><Name>F2</Name><Origin><Source>GeometricFeature</Source><FeatureName>bottom surface</FeatureName></Origin><PrimaryAxis><DefinedDirection>+Y</DefinedDirection><Source>ReferenceFrame</Source><SourceDirection>+Z</SourceDirection><FeatureName></FeatureName></PrimaryAxis><SecondaryAxis><DefinedDirection>+X</DefinedDirection><Source>ReferenceFrame</Source><SourceDirection>+Y</SourceDirection><FeatureName></FeatureName></SecondaryAxis></Value></Frame></Frames>
  wires:
  Trigonometric Function/1 -> Simulink-PS Converter/1
  Gain/1 -> Trigonometric Function/1
  Sine Wave/1 -> Gain/1
  PS-Simulink Converter/1 -> Scope/1
  Sine Wave1/1 -> Gain1/1
  Gain1/1 -> Trigonometric Function1/1
  Trigonometric Function1/1 -> Simulink-PS Converter1/1
  connections:
  World Frame/RConn1 -- Rigid Transform1/LConn1 -- Revolute Joint1/LConn1 -- Mechanism Configuration/RConn1 -- Rigid Transform/LConn1 -- Solver Configuration/RConn1
  Revolute Joint1/RConn1 -- lever horizontal/LConn1 -- lever vertical/LConn1
  linkage/LConn1 -- Spherical Joint1/LConn1
  alum extr/RConn1 -- Spherical Joint1/RConn1
  Revolute Joint1/LConn2 -- Simulink-PS Converter/RConn1
  alum extr1/RConn1 -- Spherical Joint/RConn1
  linkage1/LConn1 -- Spherical Joint/LConn1
  Revolute Joint3/RConn1 -- lever vertical1/LConn1 -- lever horizontal1/RConn1
  Simulink-PS Converter1/RConn1 -- Revolute Joint3/LConn2
  Revolute Joint3/LConn1 -- Rigid Transform1/RConn1
  Rigid Transform/RConn1 -- Spherical Joint4/LConn1
  alum extr1/LConn1 -- Spherical Joint4/RConn1 -- alum extr/LConn1 -- Rigid Transform2/LConn1
  linkage/RConn1 -- Revolute Joint/RConn1
  lever horizontal/RConn1 -- Revolute Joint/LConn1
  linkage1/RConn1 -- Spherical Joint3/RConn1
  Rigid Transform2/RConn1 -- Brick Solid/RConn1
  Spherical Joint4/RConn2 -- PS-Simulink Converter/LConn1
  lever horizontal1/LConn1 -- Spherical Joint3/LConn1
